simulink model "ControlMec"  (R2025b)
settings: Solver=VariableStepAuto  StartTime=0.0  StopTime=60  RelTol=1e-3
values from neighbouring files (symbols this model uses):
  Dm = 0.0071    [QuanserData.m]
  Dp = 0.0071    [QuanserData.m]
  Dt = 0.158    [QuanserData.m]
  g = 9.81    [QuanserData.m]
  Jeq = Jm+Jh+Jp    (= 1.120304e-05)    [QuanserData.m]
  Jp = 2.15e-2    (= 0.0215)    [QuanserData.m]
  k1 = 1.2e-5    (= 1.2e-05)    [QuanserData.m]
  k2 = 3.54e-9    (= 3.54e-09)    [QuanserData.m]
  k3 = 0    [QuanserData.m]
  k4 = 6.23e-7    (= 6.23e-07)    [QuanserData.m]
  km = 0.042    [QuanserData.m]
  Lm = 1.16e-3    (= 0.00116)    [QuanserData.m]
  Mb = 1.15    [QuanserData.m]
  Rm = 8.4    [QuanserData.m]
settings Model: Creator=y.briere  LastModifiedBy=pakaw
settings SolverCC: AlgebraicLoopSolver=TrustRegion
settings DataIOCC: InitialState=[]  LoadInitialState=on  ReturnWorkspaceOutputs=off
settings DebuggingCC: UnconnectedInputMsg=warning  UnconnectedOutputMsg=warning  UnconnectedLineMsg=warning  ArithmeticOperatorsInVariantConditions=warning
settings ModelReferenceCC: EnableRefExpFcnMdlSchedulingChecks=on
settings SFSimCC: CustomCodeUndefinedFunction=UseInterfaceOnly
settings RTWCC: GPUComputeCapability=3.5

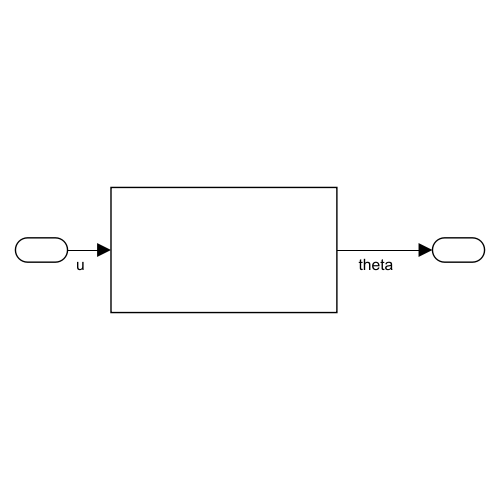
[thumbnail: Simulink's stored preview of the top-level diagram]
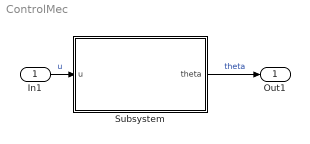
== system ControlMec ==
  In1 : Inport
  Subsystem : Subsystem
  Out1 : Outport  VectorParamsAs1DForOutWhenUnconnected=off
  wires:
  In1/1 -> Subsystem/1(u)  "u"
  Subsystem/1(theta) -> Out1/1  "theta"

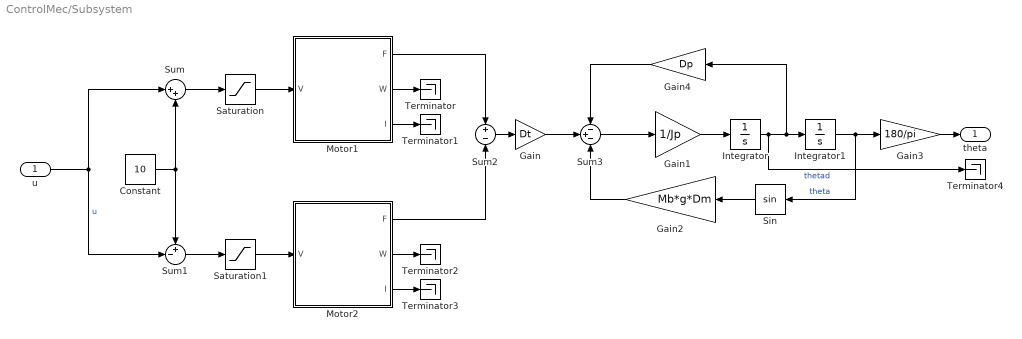
== system ControlMec/Subsystem ==
  u : Inport
  Constant : Constant  Value=10
  Gain : Gain  Gain=Dt
  Gain1 : Gain  Gain=1/Jp
  Gain2 : Gain  Gain=Mb*g*Dm
  Gain3 : Gain  Gain=180/pi
  Gain4 : Gain  Gain=Dp
  Integrator : Integrator
  Integrator1 : Integrator
  Motor1 : Subsystem
  Motor2 : Subsystem
  Saturation : Saturate  UpperLimit=24  LowerLimit=-24
  Saturation1 : Saturate  UpperLimit=24  LowerLimit=-24
  Sin : Trigonometry
  Sum : Sum  Inputs=|++
  Sum1 : Sum  Inputs=+-|
  Sum2 : Sum  Inputs=+-
  Sum3 : Sum  Inputs=-+-
  Terminator{,1..4} (5 alike) : Terminator
  theta : Outport  VectorParamsAs1DForOutWhenUnconnected=off
  wires:
  Sum2/1 -> Gain/1
  u/1 -> Sum1/2, Sum/1  "u"
  Motor1/2(W) -> Terminator/1
  Constant/1 -> Sum1/1, Sum/2
  Motor1/3(I) -> Terminator1/1
  Motor2/3(I) -> Terminator3/1
  Integrator/1 -> Terminator4/1, Gain4/1, Integrator1/1  "thetad"
  Integrator1/1 -> Gain3/1, Sin/1  "theta"
  Motor2/2(W) -> Terminator2/1
  Sum/1 -> Saturation/1
  Sum3/1 -> Gain1/1
  Gain4/1 -> Sum3/1
  Gain/1 -> Sum3/2
  Sum1/1 -> Saturation1/1
  Motor2/1(F) -> Sum2/2
  Gain1/1 -> Integrator/1
  Motor1/1(F) -> Sum2/1
  Sin/1 -> Gain2/1
  Gain2/1 -> Sum3/3
  Saturation/1 -> Motor1/1(V)
  Saturation1/1 -> Motor2/1(V)
  Gain3/1 -> theta/1

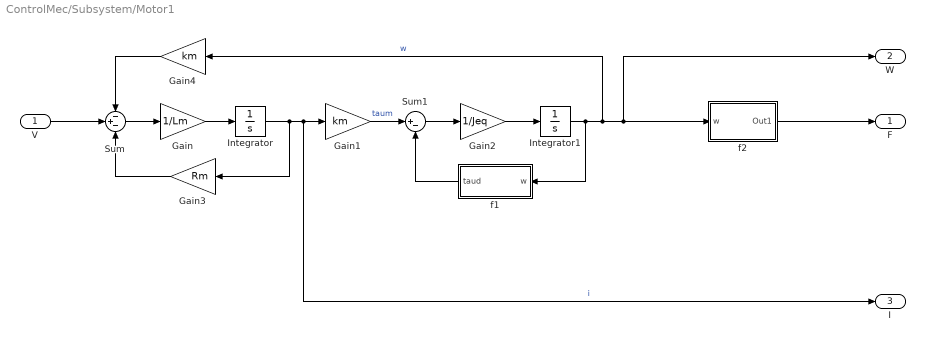
== system ControlMec/Subsystem/Motor1 ==
  V : Inport
  Gain : Gain  Gain=1/Lm
  Gain1 : Gain  Gain=km
  Gain2 : Gain  Gain=1/Jeq
  Gain3 : Gain  Gain=Rm
  Gain4 : Gain  Gain=km
  Integrator : Integrator
  Integrator1 : Integrator
  Sum : Sum  Inputs=-+-
  Sum1 : Sum  Inputs=|+-
  f1 : Subsystem
  f2 : Subsystem
  F : Outport  VectorParamsAs1DForOutWhenUnconnected=off
  W : Outport  Port=2  VectorParamsAs1DForOutWhenUnconnected=off
  I : Outport  Port=3  VectorParamsAs1DForOutWhenUnconnected=off
  wires:
  Gain4/1 -> Sum/1
  Gain/1 -> Integrator/1
  Sum1/1 -> Gain2/1
  Integrator/1 -> I/1, Gain1/1, Gain3/1  "i"
  Sum/1 -> Gain/1
  Integrator1/1 -> f1/1(w), f2/1(w), W/1, Gain4/1  "w"
  Gain3/1 -> Sum/3
  Gain1/1 -> Sum1/1  "taum"
  Gain2/1 -> Integrator1/1
  V/1 -> Sum/2
  f1/1(taud) -> Sum1/2
  f2/1(Out1) -> F/1

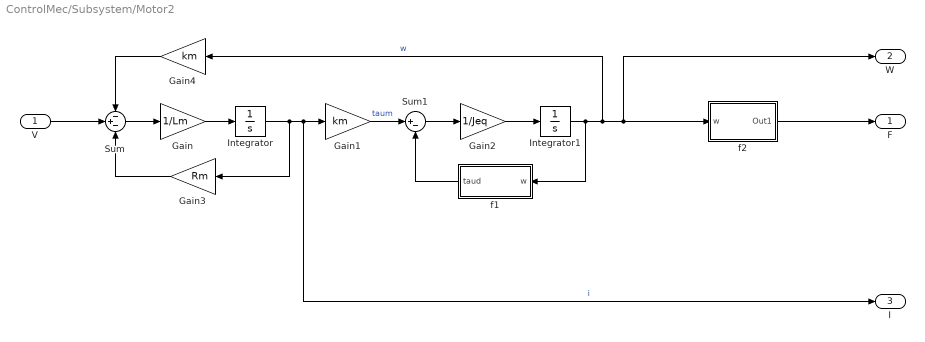
== system ControlMec/Subsystem/Motor2 ==
  V : Inport
  Gain : Gain  Gain=1/Lm
  Gain1 : Gain  Gain=km
  Gain2 : Gain  Gain=1/Jeq
  Gain3 : Gain  Gain=Rm
  Gain4 : Gain  Gain=km
  Integrator : Integrator
  Integrator1 : Integrator
  Sum : Sum  Inputs=-+-
  Sum1 : Sum  Inputs=|+-
  f1 : Subsystem
  f2 : Subsystem
  F : Outport  VectorParamsAs1DForOutWhenUnconnected=off
  W : Outport  Port=2  VectorParamsAs1DForOutWhenUnconnected=off
  I : Outport  Port=3  VectorParamsAs1DForOutWhenUnconnected=off
  wires:
  f2/1(Out1) -> F/1
  f1/1(taud) -> Sum1/2
  V/1 -> Sum/2
  Gain2/1 -> Integrator1/1
  Gain1/1 -> Sum1/1  "taum"
  Gain3/1 -> Sum/3
  Integrator1/1 -> Gain4/1, W/1, f2/1(w), f1/1(w)  "w"
  Sum/1 -> Gain/1
  Integrator/1 -> Gain3/1, Gain1/1, I/1  "i"
  Sum1/1 -> Gain2/1
  Gain/1 -> Integrator/1
  Gain4/1 -> Sum/1

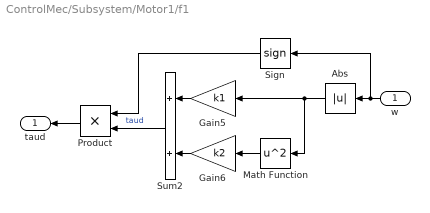
== system ControlMec/Subsystem/Motor1/f1 ==
  w : Inport
  Abs : Abs  SaturateOnIntegerOverflow=off
  Gain5 : Gain  Gain=k1
  Gain6 : Gain  Gain=k2
  Math Function : Math  Operator=square  SignedPower=on
  Product : Product
  Sign : Signum
  Sum2 : Sum
  taud : Outport
  wires:
  w/1 -> Sign/1, Abs/1
  Sum2/1 -> Product/2  "taud"
  Math Function/1 -> Gain6/1
  Gain6/1 -> Sum2/2
  Gain5/1 -> Sum2/1
  Abs/1 -> Gain5/1, Math Function/1
  Product/1 -> taud/1
  Sign/1 -> Product/1

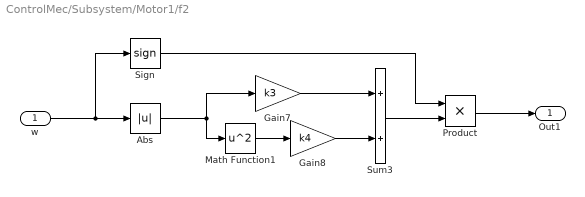
== system ControlMec/Subsystem/Motor1/f2 ==
  w : Inport
  Abs : Abs  SaturateOnIntegerOverflow=off
  Gain7 : Gain  Gain=k3
  Gain8 : Gain  Gain=k4
  Math Function1 : Math  Operator=square  SignedPower=on
  Product : Product
  Sign : Signum
  Sum3 : Sum
  Out1 : Outport
  wires:
  Gain7/1 -> Sum3/1
  Gain8/1 -> Sum3/2
  w/1 -> Sign/1, Abs/1
  Math Function1/1 -> Gain8/1
  Sum3/1 -> Product/2
  Product/1 -> Out1/1
  Abs/1 -> Gain7/1, Math Function1/1
  Sign/1 -> Product/1

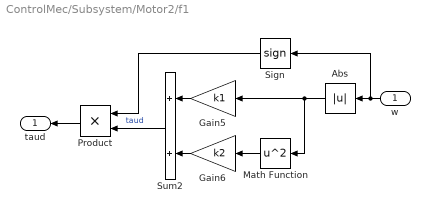
== system ControlMec/Subsystem/Motor2/f1 ==
  w : Inport
  Abs : Abs  SaturateOnIntegerOverflow=off
  Gain5 : Gain  Gain=k1
  Gain6 : Gain  Gain=k2
  Math Function : Math  Operator=square  SignedPower=on
  Product : Product
  Sign : Signum
  Sum2 : Sum
  taud : Outport
  wires:
  Sign/1 -> Product/1
  Product/1 -> taud/1
  Abs/1 -> Math Function/1, Gain5/1
  Gain5/1 -> Sum2/1
  Gain6/1 -> Sum2/2
  Math Function/1 -> Gain6/1
  Sum2/1 -> Product/2  "taud"
  w/1 -> Abs/1, Sign/1

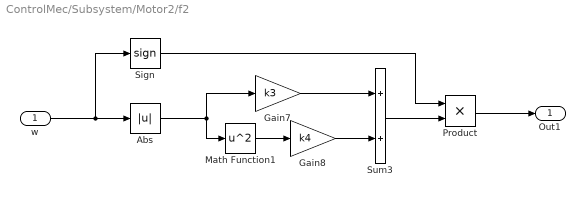
== system ControlMec/Subsystem/Motor2/f2 ==
  w : Inport
  Abs : Abs  SaturateOnIntegerOverflow=off
  Gain7 : Gain  Gain=k3
  Gain8 : Gain  Gain=k4
  Math Function1 : Math  Operator=square  SignedPower=on
  Product : Product
  Sign : Signum
  Sum3 : Sum
  Out1 : Outport
  wires:
  Sign/1 -> Product/1
  Abs/1 -> Math Function1/1, Gain7/1
  Product/1 -> Out1/1
  Sum3/1 -> Product/2
  Math Function1/1 -> Gain8/1
  w/1 -> Abs/1, Sign/1
  Gain8/1 -> Sum3/2
  Gain7/1 -> Sum3/1
